simulink model "CraneStabPiMod2"  (R2025b)
settings: Solver=ode1  StartTime=0.0  StopTime=40  FixedStep=0.001  RelTol=1e-3  EnableMultiTasking=on
model workspace (MAT data in the model file):
  PID1D = 0.2
  PID1I = 0.1
  PID1P = 5
  PIDDD = 4
  PIDDI = 0.3
  PIDDP = 8
undefined symbols (not defined in the file): MQTTsample
libraries: raspberrypiCommlib x2, raspberrypiBasiclib x1, raspberrypiIOTlib x1
settings Model: SimulationMode=external  ExtModeTrigMode=oneshot  ExtModeTrigDuration=100000  Creator=Demo11  LastModifiedBy=brfon_9d4n8nc
settings SolverCC: AlgebraicLoopSolver=TrustRegion  PositivePriorityOrder=on  AutoInsertRateTranBlk=on
settings DataIOCC: SaveFormat=Array  SignalLoggingSaveFormat=ModelDataLogs  ReturnWorkspaceOutputs=off  SignalLoggingName=sigsOut
settings OptimizationCC: BlockReduction=off  BooleanDataType=off  EnhancedBackFolding=on  PassReuseOutputArgsAs=Individual arguments  ExpressionDepthLimit=2147483647.0  ZeroExternalMemoryAtStartup=off  ZeroInternalMemoryAtStartup=off  InitFltsAndDblsToZero=on  MaxStackSize=200000  OptimizeBlockOrder=speed  DifferentSizesBufferReuse=on  OptimizationCustomize=off  EfficientTunableParamExpr=on
settings DebuggingCC: SaveWithParameterizedLinksMsg=none  UnderspecifiedInitializationDetection=Classic  MergeDetectMultiDrivingBlocksExec=none  SignalResolutionControl=TryResolveAllWithWarning  MultiTaskDSMMsg=warning  MultiTaskCondExecSysMsg=none  ParameterTunabilityLossMsg=error  FcnCallInpInsideContextMsg=warning  UnconnectedInputMsg=warning  UnconnectedOutputMsg=warning  UnconnectedLineMsg=warning  AllowSymbolicDim=off  StateNameClashWarn=warning  SFUnexpectedBacktrackingDiag=warning  SFNoUnconditionalDefaultTransitionDiag=warning  SFExecutionAtInitializationDiag=none  ArithmeticOperatorsInVariantConditions=warning
settings HardwareCC: ProdBitPerLong=64.0  ProdLargestAtomicInteger=LongLong  ProdLargestAtomicFloat=Double  ProdLongLongMode=on  ProdHWDeviceType=ARM Compatible->ARM Cortex-A (64-bit)  TargetBitPerLong=64.0  TargetBitPerPointer=64.0  TargetIntDivRoundTo=Zero  TargetEndianess=LittleEndian  TargetWordSize=64.0  TargetHWDeviceType=Intel->x86-64
settings ModelReferenceCC: EnableRefExpFcnMdlSchedulingChecks=on  PropagateSignalLabelsOutOfModel=off
settings SFSimCC: SimUseLocalCustomCode=off  CustomCodeUndefinedFunction=UseInterfaceOnly
settings RTWCC: SystemTargetFile=ert.tlc  HardwareBoard=Raspberry Pi (64bit)  TLCOptions="-aInlineSetEventsForThisBaseRateFcn=TLC_FALSE -aSuppressMultiTaskScheduler=TLC_FALSE  -aRateBasedStepFcn=0"  TemplateMakefile=ert_default_tmf  RTWUseLocalCustomCode=off  Toolchain=GNU GCC Embedded Linux  BuildConfiguration=Faster Runs  GPUComputeCapability=3.5  Description=Embedded Coder
settings CodeAppCC: ForceParamTrailComments=on  IgnoreCustomStorageClasses=off  MaxIdLength=95.0  OperatorAnnotations=on  SimulinkDataObjDesc=on  SFDataObjDesc=on  InsertBlockDesc=on
settings ERTTargetCC: ExtModeTransport=2.0  ExtModeStaticAlloc=on  ExtModeMexFile=ext_xcp  ExtModeIntrfLevel=Level2 - Open  InlinedParameterPlacement=Hierarchical  CodeReplacementLibrary=ARM Cortex-A CMSIS  SupportContinuousTime=on  SupportVariableSizeSignals=on
settings ConfigComp: CovMetricSettings=dw  CovSaveCumulativeToWorkspaceVar=on  CovSaveSingleToWorkspaceVar=on  CovExternalEMLEnable=off

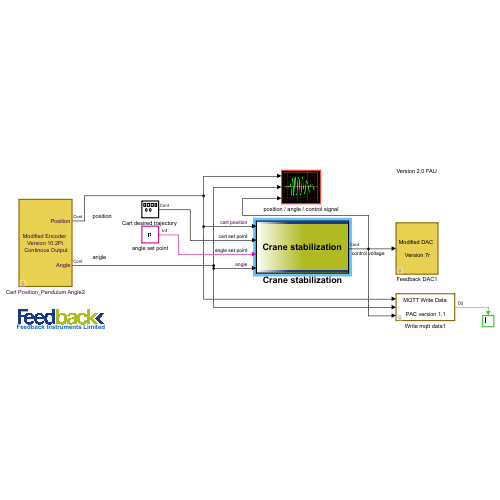
[thumbnail: Simulink's stored preview of the top-level diagram]
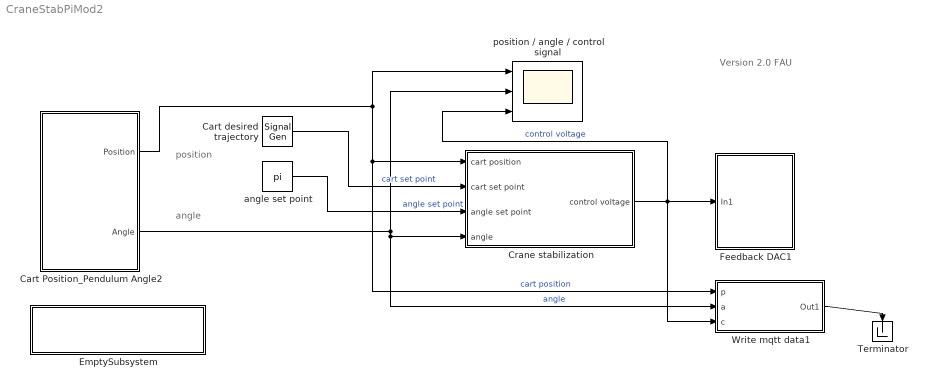
== system CraneStabPiMod2 ==
  note: position
  note: angle
  note: Version 2.0 FAU
  Cart Position_Pendulum Angle2 : Subsystem  mask(Feedback Encoder Block){st=0.001, of1=0, of2=-1024}
      mask prompts: st "Sample Time"; of1 "Channel 1 Offset"; of2 "Channel 2 Offset"
      mask help: Special block to use with the Feedback experiments to read encoder channels using the digital I/O lines
      mask Display:
      | %image(imread('bckg.bmp'))
      | disp('Modified Encoder \nVersion 10.2Pi\n Continous Output')
      | port_label('output', 1, 'Position')
      | port_label('output', 2, 'Angle')
  "Cart desired trajectory " : SignalGenerator  Amplitude=0.3  Frequency=0.1
  Crane stabilization : Subsystem
      mask Display:
      | image(imread('bckg.bmp'))
      | disp('Crane stabilization')
  EmptySubsystem : Subsystem
      mask Display:
      | image(imread('FB-inst-blue2.jpg'))
      | disp('\n\nFeedback Instruments Limited')
  Feedback DAC1 : Subsystem  mask(DAC Unit for Feedback Experiments){st=0.001, ch=1}
      mask prompts: st "Sample Time"; ch "Output Channel"
      mask help:
      | Digital to Analog Output  for Feedback Experiments
      | using Advantech PCI1711  I/O board
      mask Display:
      | %image(imread('bckg.bmp'))
      | disp('Modified DAC \n\n Version 7r')
  Terminator : Terminator
  Write mqtt data1 : Subsystem
      mask Display: disp('MQTT Write Data\n\n PAC version 1.1')
  angle set point : Constant  Value=pi
  position / angle / control signal : Scope  NumInputPorts=3
      settings: SampleTime=0.001  ActiveDisplayYMinimum=-0.55  ActiveDisplayYMaximum=0.35  DataLoggingMaxPoints=100000
      mask Display: image(imread('scope.jpg'))
  wires:
  Crane stabilization/1(control voltage) -> Write mqtt data1/3(c), Feedback DAC1/1(In1), position / angle / control signal/3  "control voltage"
  angle set point/1 -> Crane stabilization/3(angle set point)  "angle set point"
  Cart Position_Pendulum Angle2/2(Angle) -> Write mqtt data1/2(a), Crane stabilization/4(angle), position / angle / control signal/2  "angle"
  Cart Position_Pendulum Angle2/1(Position) -> Write mqtt data1/1(p), Crane stabilization/1(cart position), position / angle / control signal/1  "cart position"
  "Cart desired trajectory "/1 -> Crane stabilization/2(cart set point)  "cart set point"
  Write mqtt data1/1(Out1) -> Terminator/1

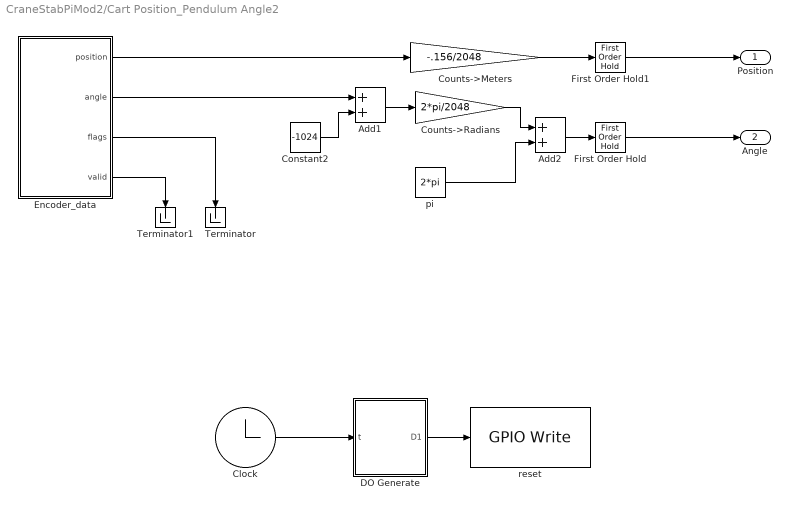
== system CraneStabPiMod2/Cart Position_Pendulum Angle2 ==
  Add1 : Sum
  Add2 : Sum
  Clock : Clock
  Constant2 : Constant  Value=-1024
  Counts->Meters : Gain  Gain=-.156/2048  SaturateOnIntegerOverflow=on  OutDataTypeStr=Inherit: Same as input  ParamDataTypeStr=Inherit: Same as input
  Counts->Radians : Gain  Gain=2*pi/2048  SaturateOnIntegerOverflow=on  OutDataTypeStr=Inherit: Same as input  ParamDataTypeStr=Inherit: Same as input
  DO Generate : MATLAB Function  TreatAsAtomicUnit=on
  Encoder_data : Subsystem
  First Order Hold : FirstOrderHold  OutputAlgorithm=Fast (Minimize Error)  ErrorTolerance=inf
  First Order Hold1 : FirstOrderHold  OutputAlgorithm=Fast (Minimize Error)  ErrorTolerance=inf
  Terminator : Terminator
  Terminator1 : Terminator
  pi : Constant  Value=2*pi
  reset : raspberrypiBasiclib/GPIO Write  BoardProperty=Pi 5 Model  gpio=6  blockPlatform=Raspberry Pi  PinNumber=17  board=[]  direction=[]
  Position : Outport
  Angle : Outport  Port=2
  wires:
  pi/1 -> Add2/2
  Counts->Radians/1 -> Add2/1
  Counts->Meters/1 -> First Order Hold1/1
  Clock/1 -> DO Generate/1(t)
  DO Generate/1(D1) -> reset/1
  Encoder_data/2(angle) -> Add1/1
  Encoder_data/1(position) -> Counts->Meters/1
  Add1/1 -> Counts->Radians/1
  Constant2/1 -> Add1/2
  Encoder_data/4(valid) -> Terminator1/1
  Encoder_data/3(flags) -> Terminator/1
  Add2/1 -> First Order Hold/1
  First Order Hold/1 -> Angle/1
  First Order Hold1/1 -> Position/1

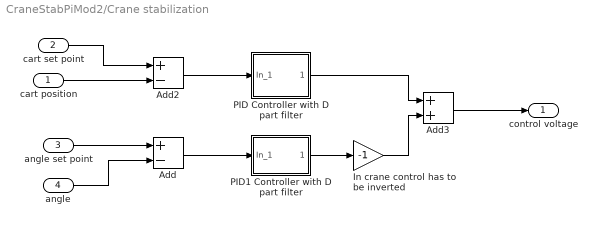
== system CraneStabPiMod2/Crane stabilization ==
  cart position : Inport
  cart set point : Inport  Port=2
  angle set point : Inport  Port=3
  angle : Inport  Port=4
  Add : Sum  Inputs=+-
  Add2 : Sum  Inputs=+-
  Add3 : Sum
  In crane control has to be inverted : Gain  Gain=-1
  PID Controller with D part filter : Subsystem  AncestorBlock=simulink_extras/Additional Linear/PID Controller  mask(PID Controller){P=PIDDP, I=PIDDI, D=PIDDD}
      mask prompts: P "Proportional:"; I "Integral:"; D "Derivative:"
      mask help:
      | Enter expressions for proportional, integral, and derivative terms.
      | P+I/s+Ds
      mask Help: This block implements a PID controller where parameters are entered for the Proportional, Integral and Derivative terms. Unmask this block to see how it works. The derivative term is implemented using a true derivative block.
      mask Callback P:
      | if str2num(get_param(gcb, 'P'))>12
      |  WARNDLG('Proportional Gain is out of the range [4..12] and is set to maximum value now', 'Setting Value Error')
      |  set_param(gcb,'P','12');
      | end
      | if str2num(get_param(gcb, 'P'))<4
      |  WARNDLG('Proportional Gain is out of the range [4..12] and is set to minimum now', 'Setting Value Error')
      |  set_param(gcb,'P','4');
      | end
      mask Callback I:
      | if str2num(get_param(gcb, 'I'))>0.5
      |  WARNDLG('Integral Gain is out of the range [0.1 .. 0.5] and is set to maximum value now', 'Setting Value Error')
      |  set_param(gcb,'I','0.5');
      | end
      | if str2num(get_param(gcb, 'I'))<0.1
      |  WARNDLG('Integral Gain is out of the range [0.1 .. 0.5] and is set to minimum now', 'Setting Value Error')
      |  set_param(gcb,'I','0.1');
      | end
      mask Callback D:
      | if str2num(get_param(gcb, 'D'))>6
      |  WARNDLG('Derivative Gain is out of the range [2..6] and is set to maximum value now', 'Setting Value Error')
      |  set_param(gcb,'D','6');
      | end
      | if str2num(get_param(gcb, 'D'))<2
      |  WARNDLG('Derivative Gain is out of the range [2..6] and is set to minimum now', 'Setting Value Error')
      |  set_param(gcb,'D','2');
      | end
      mask Display:
      | image(imread('bckg.bmp'))
      | disp('PID')
  PID1 Controller with D part filter : Subsystem  AncestorBlock=simulink_extras/Additional Linear/PID Controller  mask(PID Controller){P=PID1P, I=PID1I, D=PID1D}
      mask prompts: P "Proportional:"; I "Integral:"; D "Derivative:"
      mask help:
      | Enter expressions for proportional, integral, and derivative terms.
      | P+I/s+Ds
      mask Help: This block implements a PID controller where parameters are entered for the Proportional, Integral and Derivative terms. Unmask this block to see how it works. The derivative term is implemented using a true derivative block.
      mask Callback P:
      | if str2num(get_param(gcb, 'P'))>8
      |  WARNDLG('Proportional Gain is out of the range [2..8] and is set to maximum value now', 'Setting Value Error')
      |  set_param(gcb,'P','8');
      | end
      | if str2num(get_param(gcb, 'P'))<2
      |  WARNDLG('Proportional Gain is out of the range [2..8] and is set to minimum now', 'Setting Value Error')
      |  set_param(gcb,'P','2');
      | end
      mask Callback I:
      | if str2num(get_param(gcb, 'I'))>0.15
      |  WARNDLG('Integral Gain is out of the range [0.05 .. 0.15] and is set to maximum value now', 'Setting Value Error')
      |  set_param(gcb,'I','0.15');
      | end
      | if str2num(get_param(gcb, 'I'))<0.05
      |  WARNDLG('Integral Gain is out of the range [0.05 .. 0.15] and is set to minimum now', 'Setting Value Error')
      |  set_param(gcb,'I','0.05');
      | end
      mask Callback D:
      | if str2num(get_param(gcb, 'D'))>0.3
      |  WARNDLG('Derivative Gain is out of the range [0.1 .. 0.3] and is set to maximum value now', 'Setting Value Error')
      |  set_param(gcb,'D','0.3');
      | end
      | if str2num(get_param(gcb, 'D'))<0.1
      |  WARNDLG('Derivative Gain is out of the range [0.1 .. 0.3] and is set to minimum now', 'Setting Value Error')
      |  set_param(gcb,'D','0.1');
      | end
      mask Display:
      | image(imread('bckg.bmp'))
      | disp('PID')
  control voltage : Outport
  wires:
  angle/1 -> Add/2
  angle set point/1 -> Add/1
  cart set point/1 -> Add2/1
  cart position/1 -> Add2/2
  Add3/1 -> control voltage/1
  PID Controller with D part filter/1(Out_1) -> Add3/1
  Add2/1 -> PID Controller with D part filter/1(In_1)
  Add/1 -> PID1 Controller with D part filter/1(In_1)
  In crane control has to be inverted/1 -> Add3/2
  PID1 Controller with D part filter/1(Out_1) -> In crane control has to be inverted/1

== system CraneStabPiMod2/EmptySubsystem ==

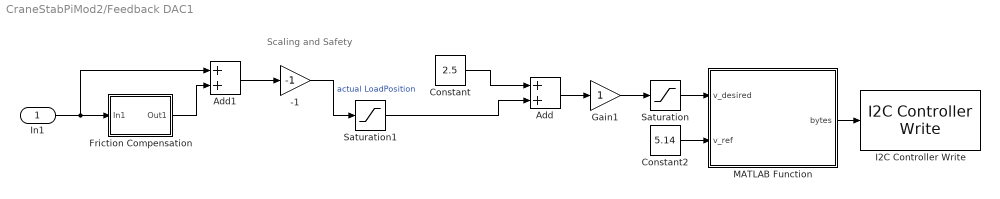
== system CraneStabPiMod2/Feedback DAC1 ==
  note: Scaling and Safety
  In1 : Inport
  -1 : Gain  Gain=-1  SaturateOnIntegerOverflow=on  OutDataTypeStr=Inherit: Same as input  ParamDataTypeStr=Inherit: Same as input
  Add : Sum  OutDataTypeStr=Inherit: Same as first input
  Add1 : Sum
  Constant : Constant  Value=2.5
  Constant2 : Constant  Value=5.14  SampleTime=-1
  Friction Compensation : Subsystem  mask(linear){frictionCompNeg=.1, frictionCompPos=.1}
      mask prompts: frictionCompNeg "Friction Compensation Magnitude in Negative Direction"; frictionCompPos "Friction Compensation Magnitude in Positive Direction"
      mask Display: plot(0,0,100,100,[40,30,20],[87,85,80],[46,54,54,46,46],[90,90,80,80,90],[46,45,45,46,54,55,55,54,46],[78,80,90,91,91,90,80,78,78],[51,51,49,49],[78,10,10,78],[90,80,70,60],[70,80,85,88],[20,10],[80,70],[20,20,15],[73,80,80],[85,80,80],[80,80,74])
  Gain1 : Gain
  I2C Controller Write : raspberrypiCommlib/I2C Controller Write  BoardProperty=Pi 5 Model  I2CModule=1  Mode=Master  SlaveAddress=0x60  SlaveByteOrder=BigEndian  Direction=Transmitter  RegisterAddressMode=off  RegisterAddress=0  SlaveDataType=uint8  DataLength=1  NoAck=off  RepeatedStart=off  OutputStatus=off
  MATLAB Function : MATLAB Function  TreatAsAtomicUnit=on
  Saturation : Saturate  UpperLimit=5.0  LowerLimit=0
  Saturation1 : Saturate  UpperLimit=2.5  LowerLimit=-2.5
  wires:
  MATLAB Function/1(bytes) -> I2C Controller Write/1
  Saturation/1 -> MATLAB Function/1(v_desired)
  Constant2/1 -> MATLAB Function/2(v_ref)
  Add1/1 -> -1/1
  -1/1 -> Saturation1/1  "actual LoadPosition"
  In1/1 -> Add1/1, Friction Compensation/1(In1)
  Friction Compensation/1(Out1) -> Add1/2
  Constant/1 -> Add/1
  Add/1 -> Gain1/1
  Gain1/1 -> Saturation/1
  Saturation1/1 -> Add/2

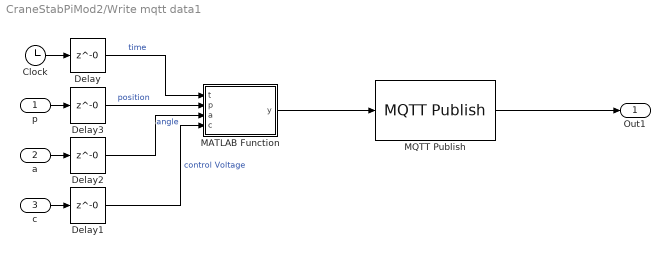
== system CraneStabPiMod2/Write mqtt data1 ==
  p : Inport
  a : Inport  Port=2
  c : Inport  Port=3
  Clock : Clock
  Delay{,1..3} (4 alike) : Delay  DelayLength=0  InitialCondition=0  SampleTime=MQTTsample
  MATLAB Function : MATLAB Function  TreatAsAtomicUnit=on
  MQTT Publish : raspberrypiIOTlib/MQTT Publish  Topic=raspi/to_django  QoS=0  RetainMsg=off  blockPlatform=RASPBERRYPI
  Out1 : Outport
  wires:
  MQTT Publish/1 -> Out1/1
  a/1 -> Delay2/1
  Clock/1 -> Delay/1
  Delay/1 -> MATLAB Function/1(t)  "time"
  p/1 -> Delay3/1
  Delay2/1 -> MATLAB Function/3(a)  "angle"
  c/1 -> Delay1/1
  Delay1/1 -> MATLAB Function/4(c)  "control Voltage"
  MATLAB Function/1(y) -> MQTT Publish/1
  Delay3/1 -> MATLAB Function/2(p)  "position"

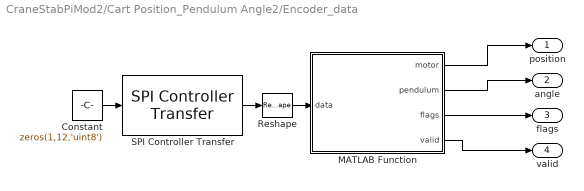
== system CraneStabPiMod2/Cart Position_Pendulum Angle2/Encoder_data ==
  Constant : Constant  Value=zeros(1,12,'uint8')
  MATLAB Function : MATLAB Function  TreatAsAtomicUnit=on
  Reshape : Reshape
  SPI Controller Transfer : raspberrypiCommlib/SPI Controller Transfer  BoardProperty=Pi 5 Model  SSPin=SPI0_CE0  SPIModule=uint32(0)  Mode=Master  BusSpeed=1000000  Pin=uint32(0)  FirstBitToTransfer=Most significant bit (MSB)  ClockMode=1  BlockFunction=Transfer  RegisterAddress=0  OutputDataType=int8  OutputDataLength=1
  position : Outport
  angle : Outport  Port=2
  flags : Outport  Port=3
  valid : Outport  Port=4
  wires:
  Constant/1 -> SPI Controller Transfer/1
  MATLAB Function/3(flags) -> flags/1
  SPI Controller Transfer/1 -> Reshape/1
  Reshape/1 -> MATLAB Function/1(data)
  MATLAB Function/2(pendulum) -> angle/1
  MATLAB Function/4(valid) -> valid/1
  MATLAB Function/1(motor) -> position/1

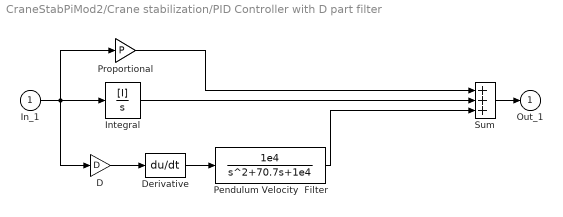
== system CraneStabPiMod2/Crane stabilization/PID Controller with D part filter ==
  In_1 : Inport
  D : Gain  Gain=D  SaturateOnIntegerOverflow=on  OutDataTypeStr=Inherit: Same as input  ParamDataTypeStr=Inherit: Same as input
  Derivative : Derivative
  Integral : TransferFcn  Numerator=[I]  Denominator=[1 0]
  Pendulum Velocity  Filter : TransferFcn  Numerator=[1e4]  Denominator=[1 70.7 1e4]
  Proportional : Gain  Gain=P  SaturateOnIntegerOverflow=on  OutDataTypeStr=Inherit: Same as input  ParamDataTypeStr=Inherit: Same as input
  Sum : Sum  Inputs=+++  InputSameDT=on  SaturateOnIntegerOverflow=on  OutDataTypeStr=Inherit: Same as first input
  Out_1 : Outport  InitialOutput=0
  wires:
  Pendulum Velocity  Filter/1 -> Sum/3
  D/1 -> Derivative/1
  Sum/1 -> Out_1/1
  In_1/1 -> Proportional/1, Integral/1, D/1
  Derivative/1 -> Pendulum Velocity  Filter/1
  Integral/1 -> Sum/2
  Proportional/1 -> Sum/1

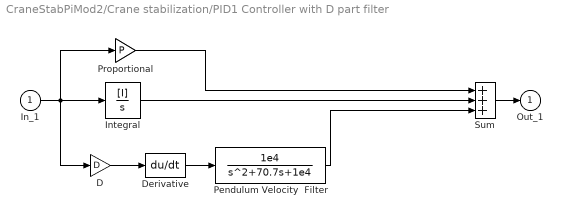
== system CraneStabPiMod2/Crane stabilization/PID1 Controller with D part filter ==
  In_1 : Inport
  D : Gain  Gain=D  SaturateOnIntegerOverflow=on  OutDataTypeStr=Inherit: Same as input  ParamDataTypeStr=Inherit: Same as input
  Derivative : Derivative
  Integral : TransferFcn  Numerator=[I]  Denominator=[1 0]
  Pendulum Velocity  Filter : TransferFcn  Numerator=[1e4]  Denominator=[1 70.7 1e4]
  Proportional : Gain  Gain=P  SaturateOnIntegerOverflow=on  OutDataTypeStr=Inherit: Same as input  ParamDataTypeStr=Inherit: Same as input
  Sum : Sum  Inputs=+++  InputSameDT=on  SaturateOnIntegerOverflow=on  OutDataTypeStr=Inherit: Same as first input
  Out_1 : Outport  InitialOutput=0
  wires:
  Proportional/1 -> Sum/1
  Integral/1 -> Sum/2
  Derivative/1 -> Pendulum Velocity  Filter/1
  In_1/1 -> Integral/1, Proportional/1, D/1
  Sum/1 -> Out_1/1
  D/1 -> Derivative/1
  Pendulum Velocity  Filter/1 -> Sum/3

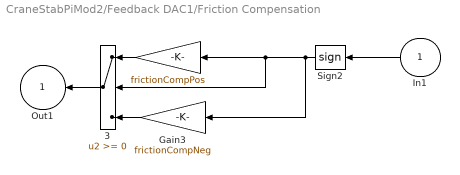
== system CraneStabPiMod2/Feedback DAC1/Friction Compensation ==
  In1 : Inport
  " " : Gain  Gain=frictionCompPos  SaturateOnIntegerOverflow=on  OutDataTypeStr=Inherit: Same as input  ParamDataTypeStr=Inherit: Same as input
  3 : Switch
  Gain3 : Gain  Gain=frictionCompNeg  SaturateOnIntegerOverflow=on  OutDataTypeStr=Inherit: Same as input  ParamDataTypeStr=Inherit: Same as input
  Sign2 : Signum  Tag=T
  Out1 : Outport  InitialOutput=0
  wires:
  3/1 -> Out1/1
  Sign2/1 -> 3/2, " "/1, Gain3/1
  Gain3/1 -> 3/3
  " "/1 -> 3/1
  In1/1 -> Sign2/1

== matlab function CraneStabPiMod2/Write mqtt data1/MATLAB Function ==
  data: t input; p input; y output; a input; c input
function y = fmtstr(t,p,a,c)

y = "{time: "+string(t)+", position: "+string(p)+", angle: "+string(a)+", control: "+string(c)+"}";

== matlab function CraneStabPiMod2/Cart Position_Pendulum Angle2/DO Generate ==
  data: D1 output; t input
%%pendulum 10
function D1  = generate_DO(t)
    if t <= 0.002
        D1 = 1;  % RESET on first sample
    else
        D1 = 0;
    end
end



%%pendulum 5
% function [D1, D2] = generate_DO(counter, t)
%     if t <= 0.002
%         D1 = 1;  % RESET on first sample
%         % D2 = 0;
%     else
%         D1 = 0;
%     %     D2 = 0;
%         % if mod(counter, 4) < 2
%         %     D1 = 0;
%         %     D2 = 0;
%         % else
%         %     D1 = 1;
%         %     D2 = 0;
%         % end
%     end
% end


%%pendulum 4
% function DO = generate_DO(counter)
%     switch counter
%         case 0
%             DO = 4;  % Reset/idle
%         case 1
%             DO = 1;  % Set DO=1 (ESP32 prepares high byte)
%         case 2
%             DO = 4;  % Keep DO=1 (Simulink reads high byte)        
%         case 3
%             DO = 4;  % Keep DO=1 (Simulink reads high byte)        
%         case 4
%             DO = 2;  % Keep DO=1 (Simulink reads high byte)        
% %         case 3
% %             DO = 1;  % Keep DO=1 (Simulink reads high byte)
% %         case 3
% %             DO = 2; %seperations
% %         case 5
% %             DO = 4; %seperations
% %         case 4
% %             DO = 2;  % Set DO=2 (ESP32 prepares low byte)
% %         case 7
% %             DO = 2;  % Keep DO=2 (Simulink reads low byte)
% %         case 8
% %             DO = 2;  % Keep DO=2 (Simulink reads low byte)
% %         case 9
% %             DO = 4;  % Unlatch
%         otherwise
%             DO = 4;
%     end
% end
% 
% function DO = generate_DO(counter)
%     % Just toggle between 0 and 1
%     if counter == 0
%         DO = 1;  % Motor state
%     else
%         DO = 0;  % Pendulum state
%     end
% end

== matlab function CraneStabPiMod2/Feedback DAC1/MATLAB Function ==
  data: v_desired input; bytes output; v_ref input
function bytes = voltToMCP4725(v_desired, v_ref)
    % v_desired: desired output voltage (0 to v_ref)
    % v_ref: DAC supply voltage (5.0)
    dacVal = uint16(round((v_desired / v_ref) * 4095));
    dacVal = min(dacVal, uint16(4095));
    b0 = uint8(64);                        % 0x40 command byte
    b1 = uint8(bitshift(dacVal, -4));      % upper 8 bits
    b2 = uint8(bitshift(bitand(dacVal, uint16(15)), 4)); % lower 4 bits
    bytes = [b0; b1; b2];
end

== matlab function CraneStabPiMod2/Cart Position_Pendulum Angle2/Encoder_data/MATLAB Function ==
  data: data input uint8 size=[1 12]; motor output; pendulum output; flags output; valid output
function [motor, pendulum, flags, valid] = unpack_spi(data)

% Checksum
chk = uint8(0);
for i = 1:9
    chk = bitxor(chk, data(i));
end
valid = logical(chk == data(10));

% Motor — bytes 1-4 little-endian
motor_int = int32(data(1)) + ...
        bitshift(int32(data(2)), 8) + ...
        bitshift(int32(data(3)), 16) + ...
        bitshift(int32(data(4)), 24);

% Pendulum — bytes 5-8 little-endian
pend_int = int32(data(5)) + ...
           bitshift(int32(data(6)), 8) + ...
           bitshift(int32(data(7)), 16) + ...
           bitshift(int32(data(8)), 24);

% Flags
flags = uint8(data(9));

% Output as single (32-bit float) for use in control blocks
motor    = double(motor_int);
pendulum = single(pend_int);

end
